simulink model "VirtualLaneSensor"  (R2026b)
settings: Solver=VariableStepAuto
undefined symbols (not defined in the file): LKA
libraries: simulink x2
settings Model: Creator=rithvin007  LastModifiedBy=rithvin007

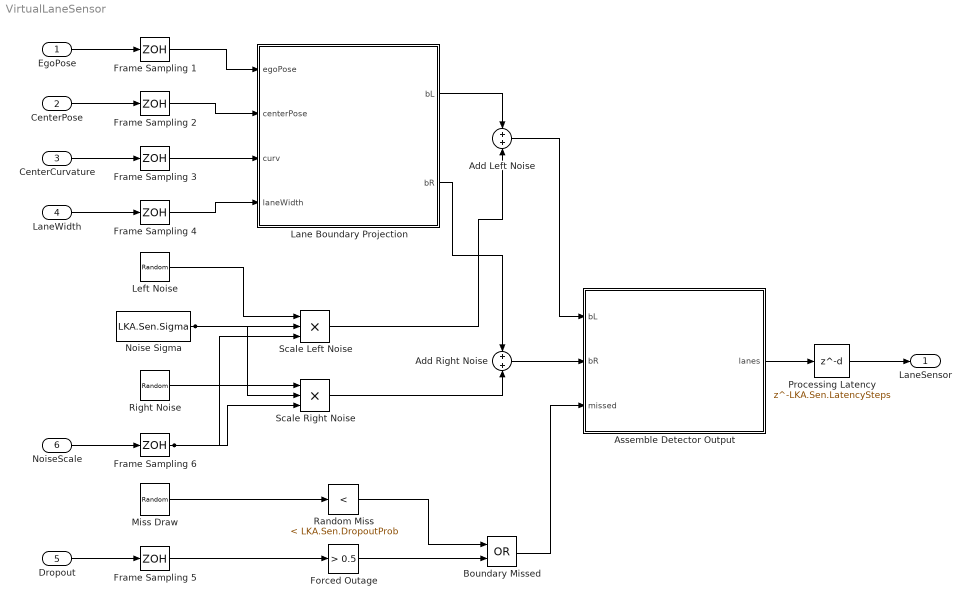
== system VirtualLaneSensor ==
  EgoPose : Inport
  CenterPose : Inport  Port=2
  CenterCurvature : Inport  Port=3
  LaneWidth : Inport  Port=4
  Dropout : Inport  Port=5
  NoiseScale : Inport  Port=6
  Add Left Noise : Sum
  Add Right Noise : Sum
  Assemble Detector Output : MATLAB Function  TreatAsAtomicUnit=on
  Boundary Missed : Logic  Operator=OR  AllPortsSameDT=off  OutDataTypeStr=boolean
  Forced Outage : simulink/Logic and Bit Operations/Compare To Constant  relop=>  const=0.5  OutDataTypeStr=boolean
  Frame Sampling {1..6} (6 alike) : ZeroOrderHold  SampleTime=LKA.Sen.Ts
  Lane Boundary Projection : MATLAB Function  TreatAsAtomicUnit=on
  Left Noise : RandomNumber  Mean=zeros(4,1)  Variance=ones(4,1)  Seed=LKA.Sen.Seed + 10 + (0:3)'  SampleTime=LKA.Sen.Ts
  Miss Draw : UniformRandomNumber  Minimum=[0;0]  Maximum=[1;1]  Seed=LKA.Sen.Seed + [40;41]  SampleTime=LKA.Sen.Ts
  Noise Sigma : Constant  Value=LKA.Sen.Sigma
  Processing Latency : Delay  DelayLength=LKA.Sen.LatencySteps  InitialCondition=0
  Random Miss : simulink/Logic and Bit Operations/Compare To Constant  relop=<  const=LKA.Sen.DropoutProb  OutDataTypeStr=boolean
  Right Noise : RandomNumber  Mean=zeros(4,1)  Variance=ones(4,1)  Seed=LKA.Sen.Seed + 20 + (0:3)'  SampleTime=LKA.Sen.Ts
  Scale Left Noise : Product  Inputs=***
  Scale Right Noise : Product  Inputs=***
  LaneSensor : Outport
  wires:
  Processing Latency/1 -> LaneSensor/1
  Assemble Detector Output/1(lanes) -> Processing Latency/1
  Add Right Noise/1 -> Assemble Detector Output/2(bR)
  Add Left Noise/1 -> Assemble Detector Output/1(bL)
  Boundary Missed/1 -> Assemble Detector Output/3(missed)
  Scale Right Noise/1 -> Add Right Noise/2
  Scale Left Noise/1 -> Add Left Noise/2
  Lane Boundary Projection/2(bR) -> Add Right Noise/1
  Frame Sampling 5/1 -> Forced Outage/1
  Miss Draw/1 -> Random Miss/1
  Frame Sampling 6/1 -> Scale Right Noise/3, Scale Left Noise/3
  CenterPose/1 -> Frame Sampling 2/1
  CenterCurvature/1 -> Frame Sampling 3/1
  LaneWidth/1 -> Frame Sampling 4/1
  Lane Boundary Projection/1(bL) -> Add Left Noise/1
  NoiseScale/1 -> Frame Sampling 6/1
  Frame Sampling 1/1 -> Lane Boundary Projection/1(egoPose)
  Forced Outage/1 -> Boundary Missed/2
  Random Miss/1 -> Boundary Missed/1
  Dropout/1 -> Frame Sampling 5/1
  Left Noise/1 -> Scale Left Noise/1
  Noise Sigma/1 -> Scale Right Noise/2, Scale Left Noise/2
  Frame Sampling 2/1 -> Lane Boundary Projection/2(centerPose)
  Frame Sampling 3/1 -> Lane Boundary Projection/3(curv)
  EgoPose/1 -> Frame Sampling 1/1
  Right Noise/1 -> Scale Right Noise/1
  Frame Sampling 4/1 -> Lane Boundary Projection/4(laneWidth)

== matlab function VirtualLaneSensor/Assemble Detector Output ==
  data: bL input; lanes output Bus: LaneSensorBus; bR input; missed input; LKA parameter
function lanes = fcn(bL, bR, missed, LKA)
% Detector message: a missed boundary is reported with strength 0
lanes.Left  = boundary(bL, ~missed(1), LKA);
lanes.Right = boundary(bR, ~missed(2), LKA);
lanes.FrameValid = true;

function b = boundary(v, seen, LKA)
if seen
    b = struct('LateralOffset', v(1), 'HeadingAngle', v(2), 'Curvature', v(3), ...
        'CurvatureDerivative', v(4), 'Strength', LKA.Sen.Strength, 'ViewRange', LKA.Sen.ViewRange);
else
    b = struct('LateralOffset', 0, 'HeadingAngle', 0, 'Curvature', 0, ...
        'CurvatureDerivative', 0, 'Strength', 0, 'ViewRange', 0);
end

== matlab function VirtualLaneSensor/Lane Boundary Projection ==
  data: egoPose input; bL output; centerPose input; curv input; laneWidth input; bR output
function [bL, bR] = fcn(egoPose, centerPose, curv, laneWidth)
% Ideal detector: lane boundaries as clothoids in the vehicle frame (see lka_lane_geometry.m)
[bL, bR] = lka_lane_geometry(egoPose(:).', centerPose(:).', curv(1), curv(2), laneWidth);
